simulink model "APSA"  (R2025b)
settings: Solver=VariableStepAuto  StartTime=0.0  StopTime=10.0  RelTol=1e-3
model workspace (MAT data in the model file):
  Baro_Interface = Simulink.Bus
  Baro_Interface.Alignment = -1
  Baro_Interface.PreserveElementDimensions = 0
  Baro_Interface.Elements_internal(1) = Simulink.BusElement
  Baro_Interface.Elements_internal(1).DimensionsMode = 'Fixed'
  Baro_Interface.Elements_internal(1).SamplingMode = 'Sample based'
  Baro_Interface.Elements_internal(1).SampleTime = -1
  Baro_Interface.Elements_internal(1).Name = 'Pressure'
  Baro_Interface.Elements_internal(1).DataType_internal = 'double'
  Baro_Interface.Elements_internal(1).Complexity = 'real'
  Baro_Interface.Elements_internal(1).Dimensions = 1
  Baro_Interface.Elements_internal(2) = Simulink.BusElement
  Baro_Interface.Elements_internal(2).DimensionsMode = 'Fixed'
  Baro_Interface.Elements_internal(2).SamplingMode = 'Sample based'
  Baro_Interface.Elements_internal(2).SampleTime = -1
  Baro_Interface.Elements_internal(2).Name = 'Temperature'
  Baro_Interface.Elements_internal(2).DataType_internal = 'double'
  Baro_Interface.Elements_internal(2).Complexity = 'real'
  Baro_Interface.Elements_internal(2).Dimensions = 1
  Baro_Interface.Elements_internal(3) = Simulink.BusElement
  Baro_Interface.Elements_internal(3).DimensionsMode = 'Fixed'
  Baro_Interface.Elements_internal(3).SamplingMode = 'Sample based'
  Baro_Interface.Elements_internal(3).SampleTime = -1
  Baro_Interface.Elements_internal(3).Name = 'Altitude'
  Baro_Interface.Elements_internal(3).DataType_internal = 'double'
  Baro_Interface.Elements_internal(3).Complexity = 'real'
  Baro_Interface.Elements_internal(3).Dimensions = 1
  Baro_Interface.DataScope = 'Auto'
  GPS_Interface = Simulink.Bus
  GPS_Interface.Alignment = -1
  GPS_Interface.PreserveElementDimensions = 0
  GPS_Interface.Elements_internal(1) = Simulink.BusElement
  GPS_Interface.Elements_internal(1).DimensionsMode = 'Fixed'
  GPS_Interface.Elements_internal(1).SamplingMode = 'Sample based'
  GPS_Interface.Elements_internal(1).SampleTime = -1
  GPS_Interface.Elements_internal(1).Name = 'Latitude'
  GPS_Interface.Elements_internal(1).DataType_internal = 'double'
  GPS_Interface.Elements_internal(1).Complexity = 'real'
  GPS_Interface.Elements_internal(1).Dimensions = 1
  GPS_Interface.Elements_internal(2) = Simulink.BusElement
  GPS_Interface.Elements_internal(2).DimensionsMode = 'Fixed'
  GPS_Interface.Elements_internal(2).SamplingMode = 'Sample based'
  GPS_Interface.Elements_internal(2).SampleTime = -1
  GPS_Interface.Elements_internal(2).Name = 'Longitude'
  GPS_Interface.Elements_internal(2).DataType_internal = 'double'
  GPS_Interface.Elements_internal(2).Complexity = 'real'
  GPS_Interface.Elements_internal(2).Dimensions = 1
  GPS_Interface.Elements_internal(3) = Simulink.BusElement
  GPS_Interface.Elements_internal(3).DimensionsMode = 'Fixed'
  GPS_Interface.Elements_internal(3).SamplingMode = 'Sample based'
  GPS_Interface.Elements_internal(3).SampleTime = -1
  GPS_Interface.Elements_internal(3).Name = 'Altitude'
  GPS_Interface.Elements_internal(3).DataType_internal = 'double'
  GPS_Interface.Elements_internal(3).Complexity = 'real'
  GPS_Interface.Elements_internal(3).Dimensions = 1
  GPS_Interface.Elements_internal(4) = Simulink.BusElement
  GPS_Interface.Elements_internal(4).DimensionsMode = 'Fixed'
  GPS_Interface.Elements_internal(4).SamplingMode = 'Sample based'
  GPS_Interface.Elements_internal(4).SampleTime = -1
  GPS_Interface.Elements_internal(4).Name = 'Fix_Status'
  GPS_Interface.Elements_internal(4).DataType_internal = 'uint8'
  GPS_Interface.Elements_internal(4).Complexity = 'real'
  GPS_Interface.Elements_internal(4).Dimensions = 1
  GPS_Interface.Elements_internal(5) = Simulink.BusElement
  GPS_Interface.Elements_internal(5).DimensionsMode = 'Fixed'
  GPS_Interface.Elements_internal(5).SamplingMode = 'Sample based'
  GPS_Interface.Elements_internal(5).SampleTime = -1
  GPS_Interface.Elements_internal(5).Name = 'Timestamp'
  GPS_Interface.Elements_internal(5).DataType_internal = 'uint32'
  GPS_Interface.Elements_internal(5).Complexity = 'real'
  GPS_Interface.Elements_internal(5).Dimensions = 1
  GPS_Interface.DataScope = 'Auto'
  IMU_Interface = Simulink.Bus
  IMU_Interface.Alignment = -1
  IMU_Interface.PreserveElementDimensions = 0
  IMU_Interface.Elements_internal(1) = Simulink.BusElement
  IMU_Interface.Elements_internal(1).DimensionsMode = 'Fixed'
  IMU_Interface.Elements_internal(1).SamplingMode = 'Sample based'
  IMU_Interface.Elements_internal(1).SampleTime = -1
  IMU_Interface.Elements_internal(1).Name = 'Accel_Y'
  IMU_Interface.Elements_internal(1).DataType_internal = 'double'
  IMU_Interface.Elements_internal(1).Complexity = 'real'
  IMU_Interface.Elements_internal(1).Dimensions = 1
  IMU_Interface.Elements_internal(2) = Simulink.BusElement
  IMU_Interface.Elements_internal(2).DimensionsMode = 'Fixed'
  IMU_Interface.Elements_internal(2).SamplingMode = 'Sample based'
  IMU_Interface.Elements_internal(2).SampleTime = -1
  IMU_Interface.Elements_internal(2).Name = 'Accel_Z'
  IMU_Interface.Elements_internal(2).DataType_internal = 'double'
  IMU_Interface.Elements_internal(2).Complexity = 'real'
  IMU_Interface.Elements_internal(2).Dimensions = 1
  IMU_Interface.Elements_internal(3) = Simulink.BusElement
  IMU_Interface.Elements_internal(3).DimensionsMode = 'Fixed'
  IMU_Interface.Elements_internal(3).SamplingMode = 'Sample based'
  IMU_Interface.Elements_internal(3).SampleTime = -1
  IMU_Interface.Elements_internal(3).Name = 'Accel_X'
  IMU_Interface.Elements_internal(3).DataType_internal = 'double'
  IMU_Interface.Elements_internal(3).Complexity = 'real'
  IMU_Interface.Elements_internal(3).Dimensions = 1
  IMU_Interface.Elements_internal(4) = Simulink.BusElement
  IMU_Interface.Elements_internal(4).DimensionsMode = 'Fixed'
  IMU_Interface.Elements_internal(4).SamplingMode = 'Sample based'
  IMU_Interface.Elements_internal(4).SampleTime = -1
  IMU_Interface.Elements_internal(4).Name = 'Gyro_Y'
  IMU_Interface.Elements_internal(4).DataType_internal = 'double'
  IMU_Interface.Elements_internal(4).Complexity = 'real'
  IMU_Interface.Elements_internal(4).Dimensions = 1
  IMU_Interface.Elements_internal(5) = Simulink.BusElement
  IMU_Interface.Elements_internal(5).DimensionsMode = 'Fixed'
  IMU_Interface.Elements_internal(5).SamplingMode = 'Sample based'
  IMU_Interface.Elements_internal(5).SampleTime = -1
  IMU_Interface.Elements_internal(5).Name = 'Gyro_Z'
  IMU_Interface.Elements_internal(5).DataType_internal = 'double'
  IMU_Interface.Elements_internal(5).Complexity = 'real'
  IMU_Interface.Elements_internal(5).Dimensions = 1
  IMU_Interface.Elements_internal(6) = Simulink.BusElement
  IMU_Interface.Elements_internal(6).DimensionsMode = 'Fixed'
  IMU_Interface.Elements_internal(6).SamplingMode = 'Sample based'
  IMU_Interface.Elements_internal(6).SampleTime = -1
  IMU_Interface.Elements_internal(6).Name = 'Gyro_X'
  IMU_Interface.Elements_internal(6).DataType_internal = 'double'
  IMU_Interface.Elements_internal(6).Complexity = 'real'
  IMU_Interface.Elements_internal(6).Dimensions = 1
  IMU_Interface.Elements_internal(7) = Simulink.BusElement
  IMU_Interface.Elements_internal(7).DimensionsMode = 'Fixed'
  IMU_Interface.Elements_internal(7).SamplingMode = 'Sample based'
  IMU_Interface.Elements_internal(7).SampleTime = -1
  IMU_Interface.Elements_internal(7).Name = 'Timestamp'
  IMU_Interface.Elements_internal(7).DataType_internal = 'uint32'
  IMU_Interface.Elements_internal(7).Complexity = 'real'
  IMU_Interface.Elements_internal(7).Dimensions = 1
  IMU_Interface.DataScope = 'Auto'
  LoRa_Interface = Simulink.Bus
  LoRa_Interface.Alignment = -1
  LoRa_Interface.PreserveElementDimensions = 0
  LoRa_Interface.Elements_internal(1) = Simulink.BusElement
  LoRa_Interface.Elements_internal(1).DimensionsMode = 'Fixed'
  LoRa_Interface.Elements_internal(1).SamplingMode = 'Sample based'
  LoRa_Interface.Elements_internal(1).SampleTime = -1
  LoRa_Interface.Elements_internal(1).Name = 'Telemetry_data'
  LoRa_Interface.Elements_internal(1).DataType_internal = 'double'
  LoRa_Interface.Elements_internal(1).Complexity = 'real'
  LoRa_Interface.Elements_internal(1).Dimensions = 1
  LoRa_Interface.Elements_internal(2) = Simulink.BusElement
  LoRa_Interface.Elements_internal(2).DimensionsMode = 'Fixed'
  LoRa_Interface.Elements_internal(2).SamplingMode = 'Sample based'
  LoRa_Interface.Elements_internal(2).SampleTime = -1
  LoRa_Interface.Elements_internal(2).Name = 'Command_Data'
  LoRa_Interface.Elements_internal(2).DataType_internal = 'uint8'
  LoRa_Interface.Elements_internal(2).Complexity = 'real'
  LoRa_Interface.Elements_internal(2).Dimensions = 1
  LoRa_Interface.Elements_internal(3) = Simulink.BusElement
  LoRa_Interface.Elements_internal(3).DimensionsMode = 'Fixed'
  LoRa_Interface.Elements_internal(3).SamplingMode = 'Sample based'
  LoRa_Interface.Elements_internal(3).SampleTime = -1
  LoRa_Interface.Elements_internal(3).Name = 'Packet_ID'
  LoRa_Interface.Elements_internal(3).DataType_internal = 'uint16'
  LoRa_Interface.Elements_internal(3).Complexity = 'real'
  LoRa_Interface.Elements_internal(3).Dimensions = 1
  LoRa_Interface.DataScope = 'Auto'
  MAG_Interface = Simulink.Bus
  MAG_Interface.Alignment = -1
  MAG_Interface.PreserveElementDimensions = 0
  MAG_Interface.Elements_internal(1) = Simulink.BusElement
  MAG_Interface.Elements_internal(1).DimensionsMode = 'Fixed'
  MAG_Interface.Elements_internal(1).SamplingMode = 'Sample based'
  MAG_Interface.Elements_internal(1).SampleTime = -1
  MAG_Interface.Elements_internal(1).Name = 'Mag_X'
  MAG_Interface.Elements_internal(1).DataType_internal = 'double'
  MAG_Interface.Elements_internal(1).Complexity = 'real'
  MAG_Interface.Elements_internal(1).Dimensions = 1
  MAG_Interface.Elements_internal(2) = Simulink.BusElement
  MAG_Interface.Elements_internal(2).DimensionsMode = 'Fixed'
  MAG_Interface.Elements_internal(2).SamplingMode = 'Sample based'
  MAG_Interface.Elements_internal(2).SampleTime = -1
  MAG_Interface.Elements_internal(2).Name = 'Mag_Y'
  MAG_Interface.Elements_internal(2).DataType_internal = 'double'
  MAG_Interface.Elements_internal(2).Complexity = 'real'
  MAG_Interface.Elements_internal(2).Dimensions = 1
  MAG_Interface.Elements_internal(3) = Simulink.BusElement
  MAG_Interface.Elements_internal(3).DimensionsMode = 'Fixed'
  MAG_Interface.Elements_internal(3).SamplingMode = 'Sample based'
  MAG_Interface.Elements_internal(3).SampleTime = -1
  MAG_Interface.Elements_internal(3).Name = 'Mag_z'
  MAG_Interface.Elements_internal(3).DataType_internal = 'double'
  MAG_Interface.Elements_internal(3).Complexity = 'real'
  MAG_Interface.Elements_internal(3).Dimensions = 1
  MAG_Interface.DataScope = 'Auto'
settings Model: Creator=spider  LastModifiedBy=spider

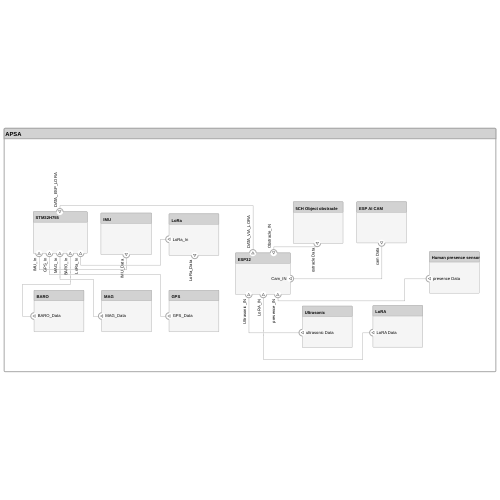
[thumbnail: Simulink's stored preview of the top-level diagram]
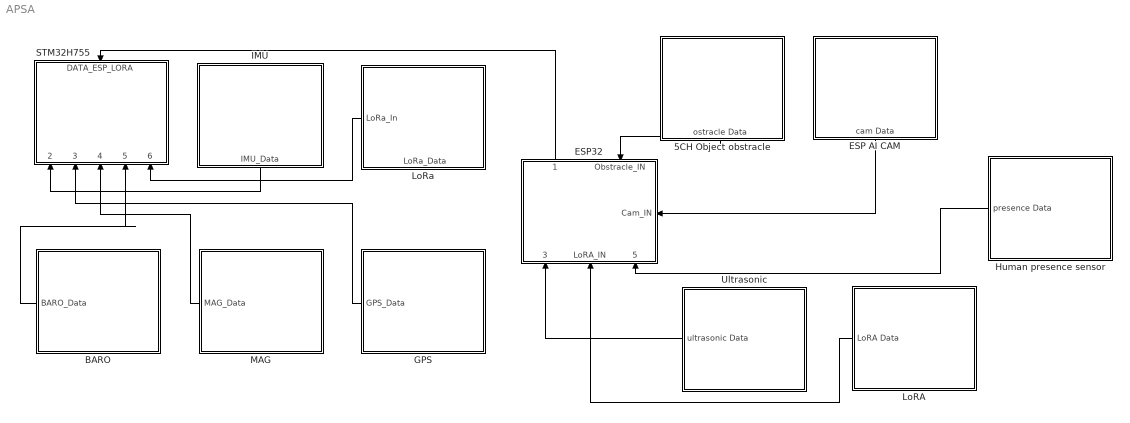
== system APSA ==
  5CH Object obstracle : Subsystem
      settings: PortSchema="{\"entries\":[{\"content\":{\"headerSize\":26,\"margin\":15,\"minimumSpacing\":25,\"sides\":[{\"content\":{},\"type\":\"ConnectorPlacement.EquallySpacedRectSide\",\"uuid\":\"6e98bced-0e35-46d5-bc8a-6741da443c36\"},{\"content\":{\"side\":\"RIGHT\"},\"type\":\"ConnectorPlacement.EquallySpacedRectSide\",\"uuid\":\"3940061c-114e-4c05-bd22-d47c5af796cd\"},{\"content\":{\"side\":\"TOP\"},\"type\":\"ConnectorPlacement.EquallySpacedRectSide\",\"uuid\":\"f7dc5be9-07bc-42bf-bc06-ffc595347593\"},{\"content\":{\"connectorIds\":[\"Out1\"],\"side\":\"BOTTOM\"},\"type\":\"ConnectorPlacement.EquallySpacedRectSide\",\"uuid\":\"504af3df-5094-436c-98d6-a89f804c981c\"}]},\"type\":\"ConnectorPlacement.EquallySpacedConnector\",\"uuid\":\"cbca699b-3ad3-47ac-92ec-d1b5aaee2861\"}],\"packageUris\":[\"http://schema.mathworks.com/mf0/Connector/R2020b\"],\"version\":\"1.0\"}"
  BARO : Subsystem
      settings: PortSchema="{\"entries\":[{\"content\":{\"headerSize\":26,\"margin\":15,\"minimumSpacing\":25,\"sides\":[{\"content\":{\"connectorIds\":[\"Out1\"]},\"type\":\"ConnectorPlacement.EquallySpacedRectSide\",\"uuid\":\"67da829c-0211-403a-929a-491a8eec0707\"},{\"content\":{\"side\":\"RIGHT\"},\"type\":\"ConnectorPlacement.EquallySpacedRectSide\",\"uuid\":\"2ec524cc-0786-49ff-83e8-dc5dc043a095\"},{\"content\":{\"side\":\"TOP\"},\"type\":\"ConnectorPlacement.EquallySpacedRectSide\",\"uuid\":\"54d38a7a-4c1b-483b-82bd-dd0984e45451\"},{\"content\":{\"side\":\"BOTTOM\"},\"type\":\"ConnectorPlacement.EquallySpacedRectSide\",\"uuid\":\"d45d699e-4c2a-4929-8b86-398358aed20d\"}]},\"type\":\"ConnectorPlacement.EquallySpacedConnector\",\"uuid\":\"1d193840-ea8e-415f-a655-00541df41638\"}],\"packageUris\":[\"http://schema.mathworks.com/mf0/Connector/R2020b\"],\"version\":\"1.0\"}"
  ESP AI CAM : Subsystem
      settings: PortSchema="{\"entries\":[{\"content\":{\"headerSize\":26,\"margin\":15,\"minimumSpacing\":25,\"sides\":[{\"content\":{},\"type\":\"ConnectorPlacement.EquallySpacedRectSide\",\"uuid\":\"6e98bced-0e35-46d5-bc8a-6741da443c36\"},{\"content\":{\"side\":\"RIGHT\"},\"type\":\"ConnectorPlacement.EquallySpacedRectSide\",\"uuid\":\"3940061c-114e-4c05-bd22-d47c5af796cd\"},{\"content\":{\"side\":\"TOP\"},\"type\":\"ConnectorPlacement.EquallySpacedRectSide\",\"uuid\":\"f7dc5be9-07bc-42bf-bc06-ffc595347593\"},{\"content\":{\"connectorIds\":[\"Out1\"],\"side\":\"BOTTOM\"},\"type\":\"ConnectorPlacement.EquallySpacedRectSide\",\"uuid\":\"cecb7cc7-9d85-4828-b1f0-9592b210c86c\"}]},\"type\":\"ConnectorPlacement.EquallySpacedConnector\",\"uuid\":\"cbca699b-3ad3-47ac-92ec-d1b5aaee2861\"}],\"packageUris\":[\"http://schema.mathworks.com/mf0/Connector/R2020b\"],\"version\":\"1.0\"}"
  ESP32 : Subsystem
      settings: PortSchema="{\"entries\":[{\"content\":{\"headerSize\":26,\"margin\":15,\"minimumSpacing\":25,\"sides\":[{\"content\":{},\"type\":\"ConnectorPlacement.EquallySpacedRectSide\",\"uuid\":\"6e98bced-0e35-46d5-bc8a-6741da443c36\"},{\"content\":{\"connectorIds\":[\"In2\"],\"side\":\"RIGHT\"},\"type\":\"ConnectorPlacement.EquallySpacedRectSide\",\"uuid\":\"3940061c-114e-4c05-bd22-d47c5af796cd\"},{\"content\":{\"connectorIds\":[\"Out1\",\"In1\"],\"side\":\"TOP\"},\"type\":\"ConnectorPlacement.EquallySpacedRectSide\",\"uuid\":\"f7dc5be9-07bc-42bf-bc06-ffc595347593\"},{\"content\":{\"connectorIds\":[\"In3\",\"In4\",\"In5\"],\"side\":\"BOTTOM\"},\"type\":\"ConnectorPlacement.EquallySpacedRectSide\",\"uuid\":\"c16906b0-a3ee-44db-b483-451e2cc0d7f8\"}]},\"type\":\"ConnectorPlacement.EquallySpacedConnector\",\"uuid\":\"cbca699b-3ad3-47ac-92ec-d1b5aaee2861\"}],\"packageUris\":[\"http://schema.mathworks.com/mf0/Connector/R2020b\"],\"version\":\"1.0\"}"
  GPS : Subsystem
      settings: PortSchema="{\"entries\":[{\"content\":{\"headerSize\":26,\"margin\":15,\"minimumSpacing\":25,\"sides\":[{\"content\":{\"connectorIds\":[\"Out1\"]},\"type\":\"ConnectorPlacement.EquallySpacedRectSide\",\"uuid\":\"67da829c-0211-403a-929a-491a8eec0707\"},{\"content\":{\"side\":\"RIGHT\"},\"type\":\"ConnectorPlacement.EquallySpacedRectSide\",\"uuid\":\"2ec524cc-0786-49ff-83e8-dc5dc043a095\"},{\"content\":{\"side\":\"TOP\"},\"type\":\"ConnectorPlacement.EquallySpacedRectSide\",\"uuid\":\"54d38a7a-4c1b-483b-82bd-dd0984e45451\"}]},\"type\":\"ConnectorPlacement.EquallySpacedConnector\",\"uuid\":\"1d193840-ea8e-415f-a655-00541df41638\"}],\"packageUris\":[\"http://schema.mathworks.com/mf0/Connector/R2020b\"],\"version\":\"1.0\"}"
  Human presence sensor : Subsystem
      settings: PortSchema="{\"entries\":[{\"content\":{\"headerSize\":26,\"margin\":15,\"minimumSpacing\":25,\"sides\":[{\"content\":{\"connectorIds\":[\"Out1\"]},\"type\":\"ConnectorPlacement.EquallySpacedRectSide\",\"uuid\":\"6e98bced-0e35-46d5-bc8a-6741da443c36\"},{\"content\":{\"side\":\"RIGHT\"},\"type\":\"ConnectorPlacement.EquallySpacedRectSide\",\"uuid\":\"3940061c-114e-4c05-bd22-d47c5af796cd\"},{\"content\":{\"side\":\"TOP\"},\"type\":\"ConnectorPlacement.EquallySpacedRectSide\",\"uuid\":\"f7dc5be9-07bc-42bf-bc06-ffc595347593\"},{\"content\":{\"side\":\"BOTTOM\"},\"type\":\"ConnectorPlacement.EquallySpacedRectSide\",\"uuid\":\"e0832bb3-6da8-4e8c-8fec-fcb53832b6df\"}]},\"type\":\"ConnectorPlacement.EquallySpacedConnector\",\"uuid\":\"cbca699b-3ad3-47ac-92ec-d1b5aaee2861\"}],\"packageUris\":[\"http://schema.mathworks.com/mf0/Connector/R2020b\"],\"version\":\"1.0\"}"
  IMU : Subsystem
      settings: PortSchema="{\"entries\":[{\"content\":{\"headerSize\":26,\"margin\":15,\"minimumSpacing\":25,\"sides\":[{\"content\":{},\"type\":\"ConnectorPlacement.EquallySpacedRectSide\",\"uuid\":\"67da829c-0211-403a-929a-491a8eec0707\"},{\"content\":{\"side\":\"RIGHT\"},\"type\":\"ConnectorPlacement.EquallySpacedRectSide\",\"uuid\":\"2ec524cc-0786-49ff-83e8-dc5dc043a095\"},{\"content\":{\"side\":\"TOP\"},\"type\":\"ConnectorPlacement.EquallySpacedRectSide\",\"uuid\":\"54d38a7a-4c1b-483b-82bd-dd0984e45451\"},{\"content\":{\"connectorIds\":[\"Out1\"],\"side\":\"BOTTOM\"},\"type\":\"ConnectorPlacement.EquallySpacedRectSide\",\"uuid\":\"6e712068-156d-43ad-ab85-0677f471e4dc\"}]},\"type\":\"ConnectorPlacement.EquallySpacedConnector\",\"uuid\":\"1d193840-ea8e-415f-a655-00541df41638\"}],\"packageUris\":[\"http://schema.mathworks.com/mf0/Connector/R2020b\"],\"version\":\"1.0\"}"
  LoRA : Subsystem
      settings: PortSchema="{\"entries\":[{\"content\":{\"headerSize\":26,\"margin\":15,\"minimumSpacing\":25,\"sides\":[{\"content\":{\"connectorIds\":[\"Out1\"]},\"type\":\"ConnectorPlacement.EquallySpacedRectSide\",\"uuid\":\"6e98bced-0e35-46d5-bc8a-6741da443c36\"},{\"content\":{\"side\":\"RIGHT\"},\"type\":\"ConnectorPlacement.EquallySpacedRectSide\",\"uuid\":\"3940061c-114e-4c05-bd22-d47c5af796cd\"},{\"content\":{\"side\":\"TOP\"},\"type\":\"ConnectorPlacement.EquallySpacedRectSide\",\"uuid\":\"f7dc5be9-07bc-42bf-bc06-ffc595347593\"},{\"content\":{\"side\":\"BOTTOM\"},\"type\":\"ConnectorPlacement.EquallySpacedRectSide\",\"uuid\":\"7c559e33-1385-47d9-a997-768beccf881e\"}]},\"type\":\"ConnectorPlacement.EquallySpacedConnector\",\"uuid\":\"cbca699b-3ad3-47ac-92ec-d1b5aaee2861\"}],\"packageUris\":[\"http://schema.mathworks.com/mf0/Connector/R2020b\"],\"version\":\"1.0\"}"
  LoRa : Subsystem
      settings: PortSchema="{\"entries\":[{\"content\":{\"headerSize\":26,\"margin\":15,\"minimumSpacing\":25,\"sides\":[{\"content\":{\"connectorIds\":[\"Out1\"]},\"type\":\"ConnectorPlacement.EquallySpacedRectSide\",\"uuid\":\"67da829c-0211-403a-929a-491a8eec0707\"},{\"content\":{\"side\":\"RIGHT\"},\"type\":\"ConnectorPlacement.EquallySpacedRectSide\",\"uuid\":\"2ec524cc-0786-49ff-83e8-dc5dc043a095\"},{\"content\":{\"side\":\"TOP\"},\"type\":\"ConnectorPlacement.EquallySpacedRectSide\",\"uuid\":\"54d38a7a-4c1b-483b-82bd-dd0984e45451\"},{\"content\":{\"connectorIds\":[\"Out2\"],\"side\":\"BOTTOM\"},\"type\":\"ConnectorPlacement.EquallySpacedRectSide\",\"uuid\":\"047cc193-b12b-4539-8571-2b3ffa899961\"}]},\"type\":\"ConnectorPlacement.EquallySpacedConnector\",\"uuid\":\"1d193840-ea8e-415f-a655-00541df41638\"}],\"packageUris\":[\"http://schema.mathworks.com/mf0/Connector/R2020b\"],\"version\":\"1.0\"}"
  MAG : Subsystem
      settings: PortSchema="{\"entries\":[{\"content\":{\"headerSize\":26,\"margin\":15,\"minimumSpacing\":25,\"sides\":[{\"content\":{\"connectorIds\":[\"Out1\"]},\"type\":\"ConnectorPlacement.EquallySpacedRectSide\",\"uuid\":\"67da829c-0211-403a-929a-491a8eec0707\"},{\"content\":{\"side\":\"RIGHT\"},\"type\":\"ConnectorPlacement.EquallySpacedRectSide\",\"uuid\":\"2ec524cc-0786-49ff-83e8-dc5dc043a095\"},{\"content\":{\"side\":\"TOP\"},\"type\":\"ConnectorPlacement.EquallySpacedRectSide\",\"uuid\":\"54d38a7a-4c1b-483b-82bd-dd0984e45451\"},{\"content\":{\"side\":\"BOTTOM\"},\"type\":\"ConnectorPlacement.EquallySpacedRectSide\",\"uuid\":\"c2529857-f248-4243-b682-7aa1651c23c3\"}]},\"type\":\"ConnectorPlacement.EquallySpacedConnector\",\"uuid\":\"1d193840-ea8e-415f-a655-00541df41638\"}],\"packageUris\":[\"http://schema.mathworks.com/mf0/Connector/R2020b\"],\"version\":\"1.0\"}"
  STM32H755 : Subsystem
      settings: PortSchema="{\"entries\":[{\"content\":{\"headerSize\":26,\"margin\":15,\"minimumSpacing\":25,\"sides\":[{\"content\":{},\"type\":\"ConnectorPlacement.EquallySpacedRectSide\",\"uuid\":\"67da829c-0211-403a-929a-491a8eec0707\"},{\"content\":{\"side\":\"RIGHT\"},\"type\":\"ConnectorPlacement.EquallySpacedRectSide\",\"uuid\":\"2ec524cc-0786-49ff-83e8-dc5dc043a095\"},{\"content\":{\"connectorIds\":[\"In1\"],\"side\":\"TOP\"},\"type\":\"ConnectorPlacement.EquallySpacedRectSide\",\"uuid\":\"54d38a7a-4c1b-483b-82bd-dd0984e45451\"},{\"content\":{\"connectorIds\":[\"In2\",\"In3\",\"In4\",\"In5\",\"In6\"],\"side\":\"BOTTOM\"},\"type\":\"ConnectorPlacement.EquallySpacedRectSide\",\"uuid\":\"9ecbcc07-50c0-4269-a635-c0099e7a9994\"}]},\"type\":\"ConnectorPlacement.EquallySpacedConnector\",\"uuid\":\"1d193840-ea8e-415f-a655-00541df41638\"}],\"packageUris\":[\"http://schema.mathworks.com/mf0/Connector/R2020b\"],\"version\":\"1.0\"}"
  Ultrasonic : Subsystem
      settings: PortSchema="{\"entries\":[{\"content\":{\"headerSize\":26,\"margin\":15,\"minimumSpacing\":25,\"sides\":[{\"content\":{\"connectorIds\":[\"Out1\"]},\"type\":\"ConnectorPlacement.EquallySpacedRectSide\",\"uuid\":\"6e98bced-0e35-46d5-bc8a-6741da443c36\"},{\"content\":{\"side\":\"RIGHT\"},\"type\":\"ConnectorPlacement.EquallySpacedRectSide\",\"uuid\":\"3940061c-114e-4c05-bd22-d47c5af796cd\"},{\"content\":{\"side\":\"TOP\"},\"type\":\"ConnectorPlacement.EquallySpacedRectSide\",\"uuid\":\"f7dc5be9-07bc-42bf-bc06-ffc595347593\"},{\"content\":{\"side\":\"BOTTOM\"},\"type\":\"ConnectorPlacement.EquallySpacedRectSide\",\"uuid\":\"bd581ea5-5fee-47b3-88cd-e83630a74304\"}]},\"type\":\"ConnectorPlacement.EquallySpacedConnector\",\"uuid\":\"cbca699b-3ad3-47ac-92ec-d1b5aaee2861\"}],\"packageUris\":[\"http://schema.mathworks.com/mf0/Connector/R2020b\"],\"version\":\"1.0\"}"
  wires:
  IMU/1(IMU_Data) -> STM32H755/2(IMU_In)
  GPS/1(GPS_Data) -> STM32H755/3(GPS_In)
  MAG/1(MAG_Data) -> STM32H755/4(MAG_In)
  BARO/1(BARO_Data) -> STM32H755/5(BARO_In)
  LoRa/1(LoRa_In) -> STM32H755/6(LoRa_In)
  5CH Object obstracle/1(ostracle Data) -> ESP32/1(Obstracle_IN)
  ESP AI CAM/1(cam Data) -> ESP32/2(Cam_IN)
  Ultrasonic/1(ultrasonic Data) -> ESP32/3(Ultrasonic_IN)
  LoRA/1(LoRA Data) -> ESP32/4(LoRA_IN)
  Human presence sensor/1(presence Data) -> ESP32/5(presence_IN)
  ESP32/1(DATA_VIA_LORA) -> STM32H755/1(DATA_ESP_LORA)

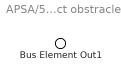
== system APSA/5CH Object obstracle ==
  Bus Element Out1 : Outport  PortName=ostracle Data

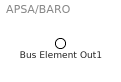
== system APSA/BARO ==
  Bus Element Out1 : Outport  PortName=BARO_Data

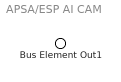
== system APSA/ESP AI CAM ==
  Bus Element Out1 : Outport  PortName=cam Data

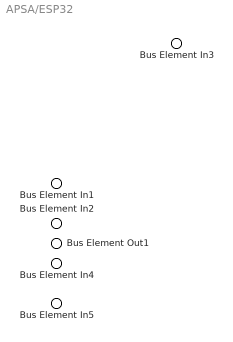
== system APSA/ESP32 ==
  Bus Element In1 : Inport  PortName=Obstracle_IN
  Bus Element In3 : Inport  Port=2  PortName=Cam_IN
  Bus Element In2 : Inport  Port=3  PortName=Ultrasonic_IN
  Bus Element In4 : Inport  Port=4  PortName=LoRA_IN
  Bus Element In5 : Inport  Port=5  PortName=presence_IN
  Bus Element Out1 : Outport  PortName=DATA_VIA_LORA

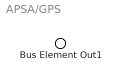
== system APSA/GPS ==
  Bus Element Out1 : Outport  PortName=GPS_Data

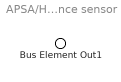
== system APSA/Human presence sensor ==
  Bus Element Out1 : Outport  PortName=presence Data

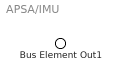
== system APSA/IMU ==
  Bus Element Out1 : Outport  PortName=IMU_Data

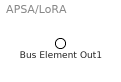
== system APSA/LoRA ==
  Bus Element Out1 : Outport  PortName=LoRA Data

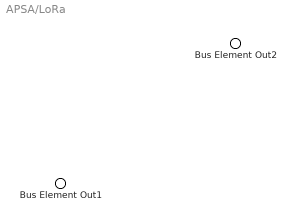
== system APSA/LoRa ==
  Bus Element Out2 : Outport  PortName=LoRa_In
  Bus Element Out1 : Outport  Port=2  PortName=LoRa_Data

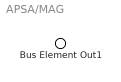
== system APSA/MAG ==
  Bus Element Out1 : Outport  PortName=MAG_Data

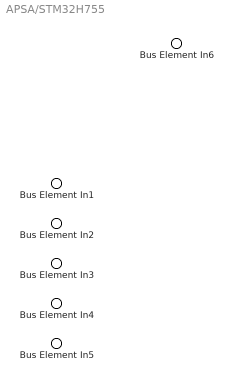
== system APSA/STM32H755 ==
  Bus Element In6 : Inport  PortName=DATA_ESP_LORA
  Bus Element In1 : Inport  Port=2  PortName=IMU_In
  Bus Element In2 : Inport  Port=3  PortName=GPS_In
  Bus Element In3 : Inport  Port=4  PortName=MAG_In
  Bus Element In4 : Inport  Port=5  PortName=BARO_In
  Bus Element In5 : Inport  Port=6  PortName=LoRa_In

== system APSA/Ultrasonic ==
  Bus Element Out1 : Outport  PortName=ultrasonic Data
